simulink model "emanuel_arc_subsystem"  (R2025a)
settings: Solver=VariableStepAuto  StartTime=0.0  StopTime=10.0  RelTol=1e-3
model workspace (MAT data in the model file):
  Rn_arc = 300
  Rp_arc = 200
  Vn_arc = 2000
  Vp_arc = 1500
libraries: spsDiodeLib x2, spsSeriesRLCBranchLib x2, spsDCVoltageSourceLib x2, spsCurrentMeasurementLib x1, spspowerguiLib x1
settings Model: Creator=hari2  LastModifiedBy=munib

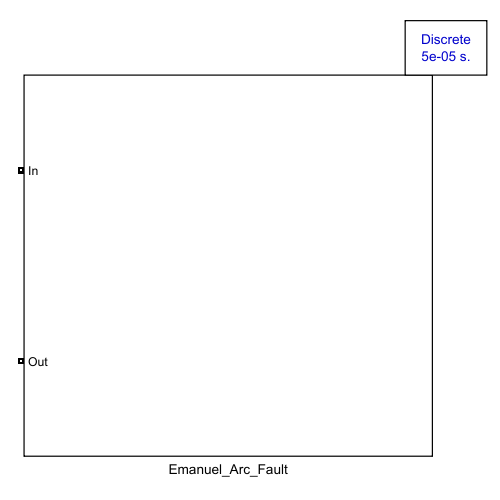
[thumbnail: Simulink's stored preview of the top-level diagram]
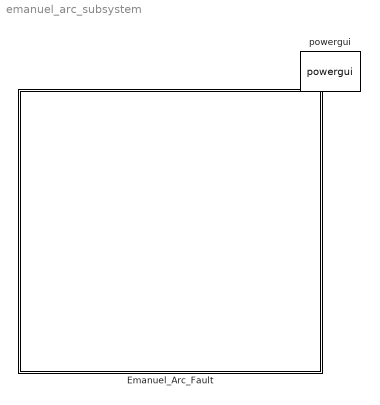
== system emanuel_arc_subsystem ==
  Emanuel_Arc_Fault : Subsystem
  powergui : spspowerguiLib/powergui  Priority=1  SimulationMode=Discrete  SampleTime=50e-6  frequency=60  Iterations=50  frequencyindice=60  Pbase=100e6  ErrMax=1e-4  UnitsV=kV  UnitsW=MW  buscounter=0  FunctionMessages=off  echomessages=off  EnableUseOfTLC=off  CurrentSourceSwitches=off  DisableSnubberDevices=off  DisableRonSwitches=off  DisableVfSwitches=off  DisplayEquations=off  AutomaticDiscreteSolvers=off  SolverType=Tustin/Backward Euler (TBE)  Interpol=off  ExternalGateDelay=off  methode=off  Ts=100  x0status=blocks  SPID=on  SwTol=0  HookPort=off  NonlinearTolerance=1e-4  nMaxIteration=100  ContinueOnMaxIteration=off  RestoreLinks=warning  ResistiveCurrentMeasurement=off  Frange=[0:2:500]  Ylog=off  Xlog=on  ShowGrid=off  save=off  variable=ZData  structure=0  ZoomFFT=off  StartTime=0.0  cycles=1  DisplayStyle=1  fundamental=60  FreqAxis=off  MaxFrequency=1000  frequencyindicesteady=1  RmsSteady=1  display=off

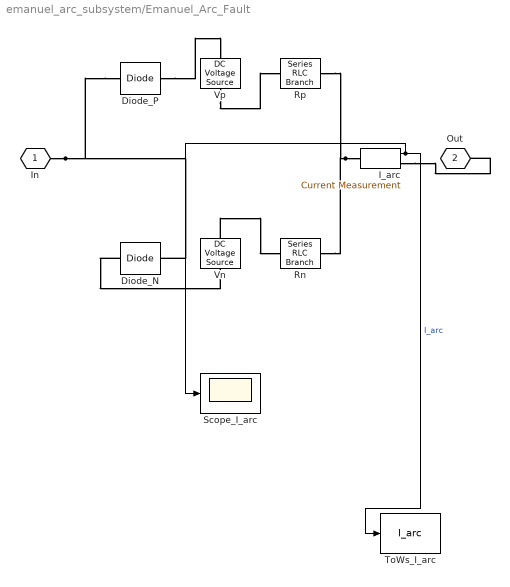
== system emanuel_arc_subsystem/Emanuel_Arc_Fault ==
  Diode_N : spsDiodeLib/Diode  Ron=0.001  Lon=0  Vf=0.8  IC=0  UseSnubber=1  Rs=1e6  Cs=inf  Measurements=off
  Diode_P : spsDiodeLib/Diode  Ron=0.001  Lon=0  Vf=0.8  IC=0  UseSnubber=1  Rs=1e6  Cs=inf  Measurements=off
  I_arc : spsCurrentMeasurementLib/Current Measurement  PhasorSimulation=off  OutputType=Complex  PSBequivalent=0
  Rn : spsSeriesRLCBranchLib/Series RLC Branch  LConnTagsString=__new0  RConnTagsString=__new0  BranchType=R  Resistance=Rn_arc  Inductance=1e-3  SetiL0=off  InitialCurrent=0  Capacitance=1e-6  Setx0=off  InitialVoltage=0  Measurements=None
  Rp : spsSeriesRLCBranchLib/Series RLC Branch  LConnTagsString=__new0  RConnTagsString=__new0  BranchType=R  Resistance=Rp_arc  Inductance=1e-3  SetiL0=off  InitialCurrent=0  Capacitance=1e-6  Setx0=off  InitialVoltage=0  Measurements=None
  Scope_I_arc : Scope
  ToWs_I_arc : ToWorkspace  VariableName=I_arc  SaveFormat=Timeseries  SampleTime=-1
  Vn : spsDCVoltageSourceLib/DC Voltage Source  Amplitude=Vn_arc  Measurements=None
  Vp : spsDCVoltageSourceLib/DC Voltage Source  Amplitude=Vp_arc  Measurements=None
  In : PMIOPort  Side=Left
  Out : PMIOPort  Port=2  Side=Left
  wires:
  I_arc/1 -> Scope_I_arc/1, ToWs_I_arc/1  "I_arc"
  connections:
  Diode_P/LConn1 -- In/RConn1 -- Diode_N/RConn1
  I_arc/LConn1 -- Rp/RConn1 -- Rn/RConn1
  Diode_N/LConn1 -- Vn/LConn1
  Vn/RConn1 -- Rn/LConn1
  I_arc/RConn1 -- Out/RConn1
  Diode_P/RConn1 -- Vp/RConn1
  Vp/LConn1 -- Rp/LConn1
